simulink model "AvonGasTurbineDgTwin_fixed"  (R2024b)
settings: Solver=VariableStepAuto  StartTime=0  StopTime=7200  FixedStep=1  RelTol=1e-3  EnableMultiTasking=on
InitFcn:
  | warning off
model workspace (MAT data in the model file):
  FAULT_01_AirIntakeFilterFouling_enable = 1
  FAULT_02_CompBladeFouling_enable = 1
  FAULT_03_CompBladeDamage_enable = 1
  FAULT_04_CompSurgeStall_enable = 1
  FAULT_05_DiffuserDamage_enable = 1
  FAULT_06_IGVStuck_enable = 1
  FAULT_07_FuelPrssRegulatorStuck_enable = 1
  FAULT_08_FuelValveLeakage_enable = 1
  FAULT_09_FuelContamination_enable = 1
  FAULT_10_FuelLineBlockage_enable = 1
  FAULT_11_FuelPumpDegradation_enable = 1
  FAULT_12_FuelSupplyPressDrop_enable = 1
  FAULT_13_FGSupplyPressOscillation_enable = 1
  FAULT_14_FGValvePartialOpening_enable = 1
  FAULT_15_FGValveActuatorDelay_enable = 1
  FAULT_15_FuelPressReg_enable = 0
  FAULT_16_CombLinerDamage_enable = 1
  FAULT_16_FuelValveLeak_enable = 0
  FAULT_17_FuelNozzleClogging_enable = 1
  FAULT_18_CombustionFlameOscillation_enable = 1
  FAULT_19_CombustionInstability_enable = 1
  FAULT_20_HotGasPathTempIncrease_enable = 1
  FAULT_21_GGTurbFouling_enable = 1
  FAULT_22_GGTurbBladeDamage_enable = 1
  FAULT_23_GGNozzleBlockage_enable = 1
  FAULT_24_GGSealDegradation_enable = 1
  FAULT_25_GGInletPressureLoss_enable = 1
  FAULT_26_PTFouling_enable = 1
  FAULT_27_PTBladeDamage_enable = 1
  FAULT_28_PTNozzleDamage_enable = 1
  FAULT_29_PTSealDegradation_enable = 1
  FAULT_30_PTBearingWear_enable = 1
  FAULT_31_PTPowerLoss_enable = 1
  FAULT_32_PTStackBlockage_enable = 1
  FAULT_33_SensorEnhancement_enable = 1
  FAULT_34_SensorDegradation_enable = 1
  FAULT_35_SensorEnhanceStep_enable = 1
  FAULT_36_SensorDegradeStep_enable = 1
  FAULT_37_SensorFreez_enable = 1
  FAULT_38_GGSpeedSensor_enable = 1
  FAULT_39_PTSpeedSensor_enable = 1
  FAULT_40_FGSensorOffset_enable = 1
  FAULT_41_FGSensorDrift_enable = 1
  FAULT_42_ControlLoopOscillation_enable = 1
  GOV_GG_BASELINE = 10
  GOV_GG_DROOP_PCT = 0.04
  GOV_PT_BASELINE = 10
  GOV_PT_DROOP_PCT = 0.04
  SW_Manual_Switch1_enable = 1
  SW_Manual_Switch2_enable = 1
  SW_Manual_Switch3_enable = 1
  SW_Manual_Switch4_enable = 1
  SW_Manual_Switch_enable = 1
undefined symbols (not defined in the file or in its folder): ENV_ambient_moisture_pct, ENV_comp_inlet_press_kPa, ENV_FG_pressure_kPa, ENV_FG_temp_C, SP_POWER_CMD
libraries: slpidlib x3, simulink x2
(part 2 of 4)

== system AvonGasTurbineDgTwin_fixed/FAULT_06_IGVStuck ==
  IGV Pos : Inport
  FAULT_06_multiplier : FromWorkspace  VariableName=FAULT_06_multiplier  SampleTime=-1
  Mux : Mux  Inputs=2
  Product : Product
  Scope{,1..3} (4 alike) : Scope  Commented=on
  Out1 : Outport
  wires:
  FAULT_06_multiplier/1 -> Product/1, Scope/1
  IGV Pos/1 -> Scope1/1, Mux/2, Product/2
  Product/1 -> Mux/1, Scope2/1, Out1/1
  Mux/1 -> Scope3/1

== system AvonGasTurbineDgTwin_fixed/FAULT_15_FuelPressReg ==
  In1 : Inport
  FAULT_15_multiplier : FromWorkspace  VariableName=FAULT_15_multiplier  SampleTime=-1
  Mux : Mux  Inputs=2
  Product : Product
  Scope{,1..3} (4 alike) : Scope  Commented=on
  Out1 : Outport
  wires:
  FAULT_15_multiplier/1 -> Product/1, Scope/1
  In1/1 -> Scope1/1, Mux/2, Product/2
  Product/1 -> Mux/1, Scope2/1, Out1/1
  Mux/1 -> Scope3/1

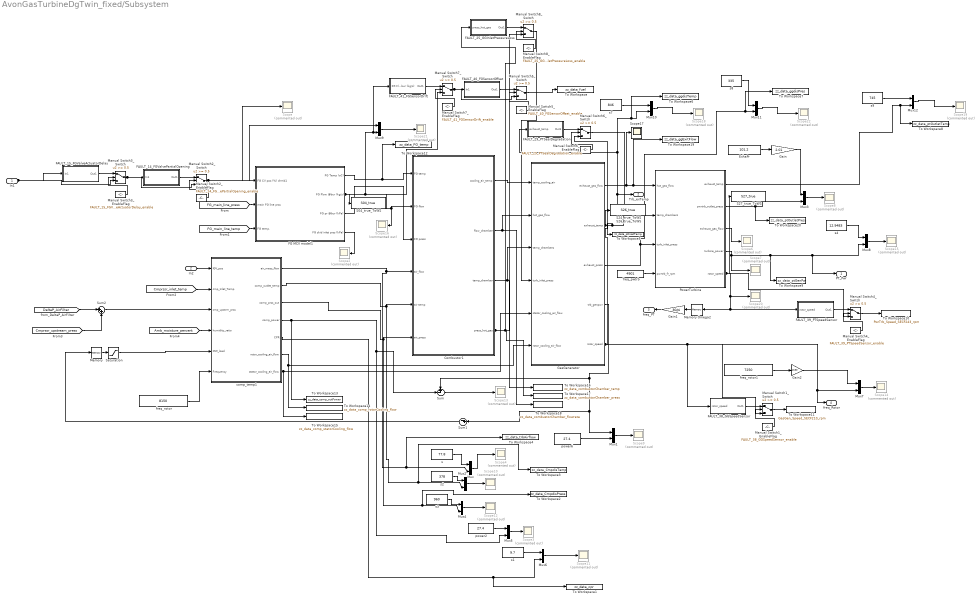
== system AvonGasTurbineDgTwin_fixed/Subsystem ==
  In1 : Inport
  In2 : Inport  Port=2
  Combustor1 : Subsystem
  ExhaPr : Constant  Value=101.2
  FAULT_14_FGValvePartialOpening : Subsystem
  FAULT_15_FGValveActuatorDelay : Subsystem
  FAULT_25_GGInletPressureLoss : Subsystem
  FAULT_29_PTSealDegradation : Subsystem
  FAULT_38_GGSpeedSensor : Subsystem
  FAULT_39_PTSpeedSensor : Subsystem
  FAULT_40_FGSensorOffset : Subsystem
  FAULT_41_FGSensorDrift : Subsystem
  FG MCV model1 : Subsystem
  Gain : Gain  Gain=2.01
  Gain1 : Gain  Gain=30/pi
  Gain2 : Gain  Gain=pi/30
  GasGenerator : Subsystem
  Manual Switch1_EnableFlag : Constant  Value=FAULT_38_GGSpeedSensor_enable
  Manual Switch1_Switch : Switch  Threshold=0.5  SaturateOnIntegerOverflow=off  InputSameDT=off
  Manual Switch2_EnableFlag : Constant  Value=FAULT_14_FGValvePartialOpening_enable
  Manual Switch2_Switch : Switch  Threshold=0.5  SaturateOnIntegerOverflow=off  InputSameDT=off
  Manual Switch3_EnableFlag : Constant  Value=FAULT_15_FGValveActuatorDelay_enable
  Manual Switch3_Switch : Switch  Threshold=0.5  SaturateOnIntegerOverflow=off  InputSameDT=off
  Manual Switch4_EnableFlag : Constant  Value=FAULT_39_PTSpeedSensor_enable
  Manual Switch4_Switch : Switch  Threshold=0.5  SaturateOnIntegerOverflow=off  InputSameDT=off
  Manual Switch5_EnableFlag : Constant  Value=FAULT_40_FGSensorOffset_enable
  Manual Switch5_Switch : Switch  Threshold=0.5  SaturateOnIntegerOverflow=off  InputSameDT=off
  Manual Switch6_EnableFlag : Constant  Value=FAULT_29_PTSealDegradation_enable
  Manual Switch6_Switch : Switch  Threshold=0.5  SaturateOnIntegerOverflow=off  InputSameDT=off
  Manual Switch7_EnableFlag : Constant  Value=FAULT_41_FGSensorDrift_enable
  Manual Switch7_Switch : Switch  Threshold=0.5  SaturateOnIntegerOverflow=off  InputSameDT=off
  Manual Switch8_EnableFlag : Constant  Value=FAULT_25_GGInletPressureLoss_enable
  Manual Switch8_Switch : Switch  Threshold=0.5  SaturateOnIntegerOverflow=off  InputSameDT=off
  Memory : Memory  InitialCondition=28.945
  Memory Omega2 : Memory  InitialCondition=pi/30*4901
  Mux{,1..12} (13 alike) : Mux  Inputs=2
  PowerTurbine : Subsystem
  S04_true_ToWS : ToWorkspace  VariableName=S04_true  SampleTime=-1
  S24_true_ToWS : ToWorkspace  VariableName=S24_true  SampleTime=-1
  S26_true_ToWS : ToWorkspace  VariableName=S26_true  SampleTime=-1
  S27_true_ToWS : ToWorkspace  VariableName=S27_true  SampleTime=-1
  Saturation : Saturate  UpperLimit=40  LowerLimit=1
  Scope{,2..4,6..16,18..22} (20 alike) : Scope  Commented=on
  Scope17 : Scope
  Sum : Sum  Inputs=+-|
  Sum1 : Sum  Inputs=-+|
  Sum2 : Sum  Inputs=|++
  To Workspace : ToWorkspace  VariableName=zz_data_fuel  SampleTime=0.2
  To Workspace1 : ToWorkspace  VariableName=zz_data_cpr  SampleTime=0.2
  To Workspace10 : ToWorkspace  VariableName=PwrTrb_Speed_SECF243_rpm  SampleTime=0.2
  To Workspace11 : ToWorkspace  VariableName=GasGen_Speed_SECF210_rpm  SampleTime=0.2
  To Workspace12 : ToWorkspace  VariableName=zz_data_FG_temp  SampleTime=0.2
  To Workspace13 : ToWorkspace  VariableName=zz_data_comp_outPower  SampleTime=0.2
  To Workspace14 : ToWorkspace  VariableName=zz_data_comp_rotorCooling_flow  SampleTime=0.2
  To Workspace15 : ToWorkspace  VariableName=zz_data_comp_statorCooling_flow  SampleTime=0.2
  To Workspace16 : ToWorkspace  VariableName=zz_data_combustorChamber_temp  SampleTime=0.2
  To Workspace17 : ToWorkspace  VariableName=zz_data_combustorChamber_press  SampleTime=0.2
  To Workspace18 : ToWorkspace  VariableName=zz_data_combustorChamber_flowrate  SampleTime=0.2
  To Workspace19 : ToWorkspace  VariableName=zz_data_ggExitFlow  SampleTime=0.2
  To Workspace2 : ToWorkspace  VariableName=zz_data_CmpdisPress  SampleTime=0.2
  To Workspace20 : ToWorkspace  VariableName=zz_data_ptOutletPress  SampleTime=0.2
  To Workspace3 : ToWorkspace  VariableName=zz_data_CmpdisTemp  SampleTime=0.2
  To Workspace4 : ToWorkspace  VariableName=zz_data_trbAirflow  SampleTime=0.2
  To Workspace5 : ToWorkspace  VariableName=zz_data_ptInletTemp  SampleTime=0.2
  To Workspace6 : ToWorkspace  VariableName=zz_data_ggdisTemp  SampleTime=0.2
  To Workspace7 : ToWorkspace  VariableName=zz_data_ggdisPres  SampleTime=0.2
  To Workspace8 : ToWorkspace  VariableName=zz_data_ptOutletTemp  SampleTime=0.2
  To Workspace9 : ToWorkspace  VariableName=zz_data_ptGenPw  SampleTime=0.2
  comp_temp1 : Subsystem
  freq_pwtrb : Constant  Value=4901
  freq_rotor : Constant  Value=8150
  freq_rotor1 : Constant  Value=7250
  power2 : Constant  Value=27.4
  power6 : Constant  Value=27.4
  s : Constant  Value=77.8
  s1 : Constant  Value=9.7
  s2 : Constant  Value=378
  s3 : Constant  Value=960
  s4 : Constant  Value=12.9483
  s7 : Constant  Value=846
  s8 : Constant  Value=335
  s9 : Constant  Value=745
  PT_Pwr : Outport
  Trb_exTemp : Outport  Port=2
  freq_PT : Outport  Port=3
  freq_Rotor : Outport  Port=4
  wires:
  Gain1/1 -> freq_PT/1
  GasGenerator/2(exhaust_temp) -> To Workspace5/1, Trb_exTemp/1, To Workspace6/1, Mux10/2, FAULT_29_PTSealDegradation/1(exhaust_temp), Manual Switch6_Switch/3, S26_true_ToWS/1
  [Amb_moisture_percent] -> comp_temp1/4(humidity_ratio)
  freq_rotor/1 -> comp_temp1/6(Frequency)
  In2/1 -> comp_temp1/1(IGV_pos)
  PowerTurbine/3(exhaust_gas_flow) -> Scope6/1
  Memory/1 -> Saturation/1
  comp_temp1/3(comp_prss_out) -> To Workspace2/1, Mux4/2, Combustor1/6(air_press)
  FG MCV model1/2(FG Flow @bur (kg/s)) -> Mux9/2, FAULT_41_FGSensorDrift/1(FG Flow @bur (kg/s)), Scope16/1, Combustor1/2(FG flow), Manual Switch7_Switch/3, S04_true_ToWS/1
  Combustor1/2(flow_chamber) -> To Workspace18/1, GasGenerator/2(hot_gas_flow)
  comp_temp1/4(comp_power) -> To Workspace13/1, Mux5/2, Sum/2
  Mux1/1 -> Scope9/1
  Mux6/1 -> Scope11/1
  comp_temp1/5(CPR) -> To Workspace1/1, Mux6/2
  Mux4/1 -> Scope12/1
  FG MCV model1/1(FG Temp (oC)) -> To Workspace12/1, Combustor1/1(FG temp)
  Mux2/1 -> Scope10/1
  [FG_main_line_press] -> FG MCV model1/2(main FG line prss)
  ExhaPr/1 -> Gain/1
  Combustor1/1(cooling_air_temp) -> GasGenerator/1(temp_cooling_air)
  FG MCV model1/3(FG pr @bur (kPa)) -> Combustor1/3(FG press)
  GasGenerator/3(exhaust_press) -> To Workspace7/1, Mux11/2, PowerTurbine/3(turb_inlet_press)
  Combustor1/3(temp_chamber) -> To Workspace16/1, GasGenerator/3(temp_chambers)
  FG MCV model1/4(FG skid inlet prss (kPa)) -> Scope2/1
  GasGenerator/1(exhaust_gas_flow) -> Scope17/1, To Workspace19/1, PowerTurbine/1(hot_gas_flow)
  PowerTurbine/2(pwrtrb_outlet_press) -> To Workspace20/1, Mux3/2
  power6/1 -> Mux1/2
  Gain/1 -> Mux3/1
  Mux3/1 -> Scope8/1
  comp_temp1/1(air_mass_flow) -> To Workspace4/1, Mux/2, Combustor1/4(air_flow)
  PowerTurbine/1(exhaust_temp) -> To Workspace8/1, Mux12/2
  comp_temp1/2(comp_outlet_temp) -> To Workspace3/1, Mux2/2, Combustor1/5(air temp)
  Mux8/1 -> Scope15/1
  Mux7/1 -> Scope14/1
  In1/1 -> FAULT_15_FGValveActuatorDelay/1(In1), Manual Switch3_Switch/3
  PowerTurbine/4(turbine_power) -> To Workspace9/1, PT_Pwr/1, Mux8/2, Scope7/1
  comp_temp1/7(stator_cooling_air_flow) -> GasGenerator/5(stator_cooling_air_flow), To Workspace15/1
  [Cmprssr_inlet_temp] -> comp_temp1/2(cmp_Inlet_Temp)
  Mux11/1 -> Scope22/1
  s2/1 -> Mux2/1
  Sum1/1 -> Memory/1
  Mux9/1 -> Scope21/1
  Mux/1 -> Scope4/1
  s/1 -> Mux/1
  s7/1 -> Mux10/1
  s1/1 -> Mux6/1
  Mux10/1 -> Scope18/1
  Mux5/1 -> Scope3/1
  Sum/1 -> Scope13/1
  GasGenerator/5(rotor_speed) -> freq_Rotor/1, Mux7/2, FAULT_38_GGSpeedSensor/1(rotor_speed), Manual Switch1_Switch/3, S24_true_ToWS/1
  comp_temp1/6(rotor_cooling_air_flow) -> GasGenerator/6(rotor_cooling_air_flow), To Workspace14/1
  s3/1 -> Mux4/1
  freq_pwtrb/1 -> PowerTurbine/4(pwrtrb_fr_rpm)
  power2/1 -> Mux5/1
  PowerTurbine/5(rotor_speed) -> Memory Omega2/1, FAULT_39_PTSpeedSensor/1(rotor_speed), Scope20/1, Manual Switch4_Switch/3, S27_true_ToWS/1
  Gain2/1 -> Mux7/1
  Saturation/1 -> comp_temp1/5(MW_load)
  Memory Omega2/1 -> Gain1/1
  freq_rotor1/1 -> Gain2/1
  GasGenerator/4(trb_genpwr) -> Sum/1, Sum1/2, Mux1/1
  s4/1 -> Mux8/1
  s9/1 -> Mux12/1
  s8/1 -> Mux11/1
  Mux12/1 -> Scope19/1
  [FG_main_line_temp] -> FG MCV model1/3(FG temp.)
  [DeltaP_AirFilter] -> Sum2/1
  [Cmprssr_upstream_press] -> Sum2/2
  Sum2/1 -> comp_temp1/3(cmp_upstrm_prss)
  Combustor1/4(press_hot_gas) -> To Workspace17/1, FAULT_25_GGInletPressureLoss/1(press_hot_gas), Manual Switch8_Switch/3
  FAULT_38_GGSpeedSensor/1(Out1) -> Manual Switch1_Switch/1
  Manual Switch1_EnableFlag/1 -> Manual Switch1_Switch/2
  Manual Switch1_Switch/1 -> To Workspace11/1
  FAULT_14_FGValvePartialOpening/1(Out1) -> Manual Switch2_Switch/1
  Manual Switch2_EnableFlag/1 -> Manual Switch2_Switch/2
  Manual Switch2_Switch/1 -> FG MCV model1/1(FG CV pos (%) chmb1), Scope/1, Mux9/1
  FAULT_15_FGValveActuatorDelay/1(Out1) -> Manual Switch3_Switch/1
  Manual Switch3_EnableFlag/1 -> Manual Switch3_Switch/2
  Manual Switch3_Switch/1 -> Manual Switch2_Switch/3, FAULT_14_FGValvePartialOpening/1(In1)
  FAULT_39_PTSpeedSensor/1(Out1) -> Manual Switch4_Switch/1
  Manual Switch4_EnableFlag/1 -> Manual Switch4_Switch/2
  Manual Switch4_Switch/1 -> To Workspace10/1
  FAULT_40_FGSensorOffset/1(Out1) -> Manual Switch5_Switch/1
  Manual Switch5_EnableFlag/1 -> Manual Switch5_Switch/2
  Manual Switch5_Switch/1 -> To Workspace/1
  FAULT_29_PTSealDegradation/1(Out1) -> Manual Switch6_Switch/1
  Manual Switch6_EnableFlag/1 -> Manual Switch6_Switch/2
  Manual Switch6_Switch/1 -> PowerTurbine/2(temp_chambers)
  FAULT_41_FGSensorDrift/1(Out1) -> Manual Switch7_Switch/1
  Manual Switch7_EnableFlag/1 -> Manual Switch7_Switch/2
  Manual Switch7_Switch/1 -> Manual Switch5_Switch/3, FAULT_40_FGSensorOffset/1(In1)
  FAULT_25_GGInletPressureLoss/1(Out1) -> Manual Switch8_Switch/1
  Manual Switch8_EnableFlag/1 -> Manual Switch8_Switch/2
  Manual Switch8_Switch/1 -> GasGenerator/4(turb_inlet_press)

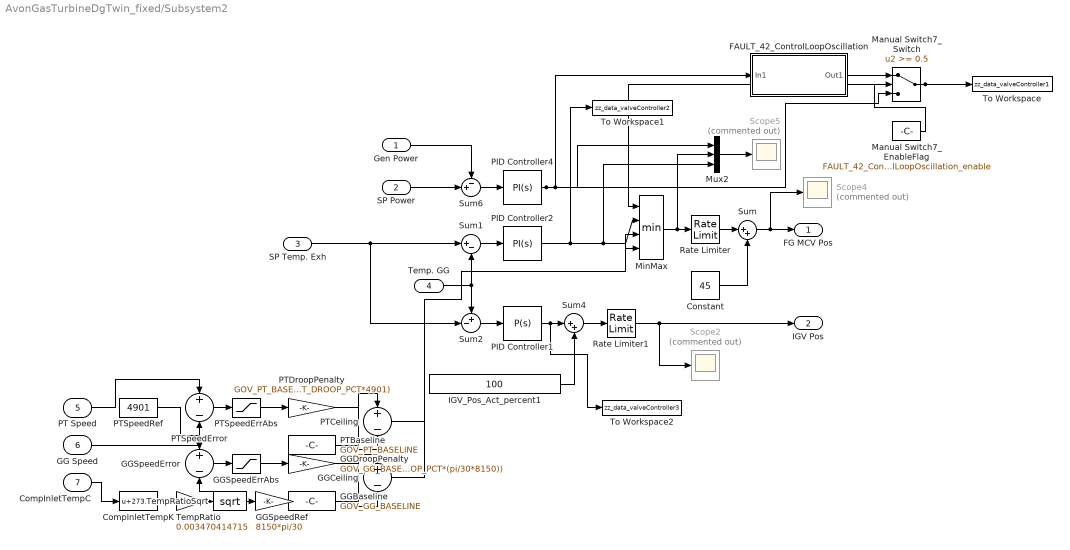
== system AvonGasTurbineDgTwin_fixed/Subsystem2 ==
  Gen Power : Inport
  SP Power : Inport  Port=2
  SP Temp. Exh : Inport  Port=3
  Temp. GG : Inport  Port=4
  PT Speed : Inport  Port=5
  GG Speed : Inport  Port=6
  CompInletTempC : Inport  Port=7
  CompInletTempK : Bias  Bias=273.15  SaturateOnIntegerOverflow=off
  Constant : Constant  Value=45
  FAULT_42_ControlLoopOscillation : Subsystem
  GGBaseline : Constant  Value=GOV_GG_BASELINE
  GGCeiling : Sum  Inputs=+-
  GGDroopPenalty : Gain  Gain=GOV_GG_BASELINE/(GOV_GG_DROOP_PCT*(pi/30*8150))
  GGSpeedErrAbs : Saturate  UpperLimit=Inf  LowerLimit=0
  GGSpeedError : Sum  Inputs=+-
  GGSpeedRef : Gain  Gain=8150*pi/30
  IGV_Pos_Act_percent1 : Constant  Value=100
  Manual Switch7_EnableFlag : Constant  Value=FAULT_42_ControlLoopOscillation_enable
  Manual Switch7_Switch : Switch  Threshold=0.5  SaturateOnIntegerOverflow=off  InputSameDT=off
  MinMax : MinMax  Inputs=4
  Mux2 : Mux  Inputs=3
  PID Controller1 : slpidlib/PID Controller  Controller=P  Form=Ideal  TimeDomain=Continuous-time  UseExternalTs=off  SampleTime=-1  IntegratorMethod=Forward Euler  FilterMethod=Forward Euler  ControllerParametersSource=internal  P=0.1  I=0.180070827922895  UseKiTs=off  D=0  UseExternalDerivativeSource=off  N=100  UseFilter=on  TunerSelectOption=Transfer Function Based (PID Tuner App)  InitialConditionSource=internal  InitialConditionForIntegrator=0  InitialConditionForFilter=0  DifferentiatorICPrevScaledInput=0  ExternalReset=none  TrackingMode=off  Kt=1  LimitOutput=on  SatLimitsSource=internal  UpperSaturationLimit=15  LowerSaturationLimit=-100  LinearizeAsGain=on  AntiWindupMode=back-calculation  Kb=0.2  LimitIntegrator=off  UpperIntegratorSaturationLimit=inf  LowerIntegratorSaturationLimit=-inf  POutMin=[]  POutMax=[]  IOutMin=[]  IOutMax=[]  DOutMin=[]  DOutMax=[]  NOutMin=[]  NOutMax=[]  SumOutMin=[]  SumOutMax=[]  SaturationOutMin=[]  SaturationOutMax=[]  PParamMin=[]  PParamMax=[]  IParamMin=[]  IParamMax=[]  DParamMin=[]  DParamMax=[]  NParamMin=[]  NParamMax=[]  KbParamMin=[]  KbParamMax=[]  KtParamMin=[]  KtParamMax=[]  KbOutMin=[]  KbOutMax=[]  KtOutMin=[]  KtOutMax=[]  IntegratorOutMin=[]  IntegratorOutMax=[]  FilterOutMin=[]  FilterOutMax=[]  SumI1OutMin=[]  SumI1OutMax=[]  SumI2OutMin=[]  SumI2OutMax=[]  SumI3OutMin=[]  SumI3OutMax=[]  SumI4OutMin=[]  SumI4OutMax=[]  SumDOutMin=[]  SumDOutMax=[]  DifferentiatorOutMin=[]  DifferentiatorOutMax=[]  FilterDiffOutCoefMin=[]  FilterDiffOutCoefMax=[]  ReciprocalOutMin=[]  ReciprocalOutMax=[]  SumDenOutMin=[]  SumDenOutMax=[]  SumNumOutMin=[]  SumNumOutMax=[]  DivideOutMin=[]  DivideOutMax=[]  UdiffTsProdOutMin=[]  UdiffTsProdOutMax=[]  NTsProdOutMin=[]  NTsProdOutMax=[]  UintegralTsProdOutMin=[]  UintegralTsProdOutMax=[]  UngainTsProdOutMin=[]  UngainTsProdOutMax=[]  ClampingZeroOutDataTypeStr=Inherit: Inherit via back propagation  ClampingZeroOutMin=[]  ClampingZeroOutMax=[]  FilterDenConstantOutDataTypeStr=Inherit: Inherit via back propagation  FilterDenConstantOutMin=[]  FilterDenConstantOutMax=[]  PCopyOutDataTypeStr=Inherit: Inherit via back propagation  PCopyOutMin=[]  PCopyOutMax=[]  NCopyOutDataTypeStr=Inherit: Inherit via back propagation  NCopyOutMin=[]  NCopyOutMax=[]  IntegratorContinuousStateAttributes=''  IntegratorStateMustResolveToSignalObject=off  IntegratorRTWStateStorageClass=Auto  FilterContinuousStateAttributes=''  FilterStateMustResolveToSignalObject=off  FilterRTWStateStorageClass=Auto  ParallelPVariant=InternalParameters  IdealPVariant=Disabled  IVariant=Disabled  DVariant=Disabled  IntegratorVariant=Disabled  SatVariant=Enabled  AWVariant=Disabled  PCopyVariant=Disabled  TRVariant=Disabled  FdbkBlocksVariant=Forward  IdealPFdbkVariant=Disabled  SatFdbkVariant=Disabled  DerivativeFilterVariant=Disabled  NVariant=Disabled  NCopyVariant=Disabled_SignalSpec  FilterICVariant=Disabled  IntegratorICVariant=Disabled  ExternalResetVariant=Disabled  TRSumVariant=Passthrough  SumFdbkVariant=Disabled  SumVariant=Passthrough_P  TsampFilterVariant=InternalTs  TsampNgainVariant=Passthrough  TsampIntegralVariant=Disabled_SignalSpec  ExternalSaturationOutDataTypeStr=Inherit: Same as second input  DerivativeSourceVariant=Disabled  PreIntVariant=InternalPreInt
  PID Controller2 : slpidlib/PID Controller  Controller=PI  Form=Ideal  TimeDomain=Continuous-time  UseExternalTs=off  SampleTime=-1  IntegratorMethod=Forward Euler  FilterMethod=Forward Euler  ControllerParametersSource=internal  P=0.02  I=0.1  UseKiTs=off  D=0  UseExternalDerivativeSource=off  N=100  UseFilter=on  TunerSelectOption=Transfer Function Based (PID Tuner App)  InitialConditionSource=internal  InitialConditionForIntegrator=20  InitialConditionForFilter=0  DifferentiatorICPrevScaledInput=0  ExternalReset=none  TrackingMode=off  Kt=1  LimitOutput=on  SatLimitsSource=internal  UpperSaturationLimit=45  LowerSaturationLimit=-45  LinearizeAsGain=on  AntiWindupMode=back-calculation  Kb=0.2  LimitIntegrator=off  UpperIntegratorSaturationLimit=inf  LowerIntegratorSaturationLimit=-inf  POutMin=[]  POutMax=[]  IOutMin=[]  IOutMax=[]  DOutMin=[]  DOutMax=[]  NOutMin=[]  NOutMax=[]  SumOutMin=[]  SumOutMax=[]  SaturationOutMin=[]  SaturationOutMax=[]  PParamMin=[]  PParamMax=[]  IParamMin=[]  IParamMax=[]  DParamMin=[]  DParamMax=[]  NParamMin=[]  NParamMax=[]  KbParamMin=[]  KbParamMax=[]  KtParamMin=[]  KtParamMax=[]  KbOutMin=[]  KbOutMax=[]  KtOutMin=[]  KtOutMax=[]  IntegratorOutMin=[]  IntegratorOutMax=[]  FilterOutMin=[]  FilterOutMax=[]  SumI1OutMin=[]  SumI1OutMax=[]  SumI2OutMin=[]  SumI2OutMax=[]  SumI3OutMin=[]  SumI3OutMax=[]  SumI4OutMin=[]  SumI4OutMax=[]  SumDOutMin=[]  SumDOutMax=[]  DifferentiatorOutMin=[]  DifferentiatorOutMax=[]  FilterDiffOutCoefMin=[]  FilterDiffOutCoefMax=[]  ReciprocalOutMin=[]  ReciprocalOutMax=[]  SumDenOutMin=[]  SumDenOutMax=[]  SumNumOutMin=[]  SumNumOutMax=[]  DivideOutMin=[]  DivideOutMax=[]  UdiffTsProdOutMin=[]  UdiffTsProdOutMax=[]  NTsProdOutMin=[]  NTsProdOutMax=[]  UintegralTsProdOutMin=[]  UintegralTsProdOutMax=[]  UngainTsProdOutMin=[]  UngainTsProdOutMax=[]  ClampingZeroOutDataTypeStr=Inherit: Inherit via back propagation  ClampingZeroOutMin=[]  ClampingZeroOutMax=[]  FilterDenConstantOutDataTypeStr=Inherit: Inherit via back propagation  FilterDenConstantOutMin=[]  FilterDenConstantOutMax=[]  PCopyOutDataTypeStr=Inherit: Inherit via back propagation  PCopyOutMin=[]  PCopyOutMax=[]  NCopyOutDataTypeStr=Inherit: Inherit via back propagation  NCopyOutMin=[]  NCopyOutMax=[]  IntegratorContinuousStateAttributes=''  IntegratorStateMustResolveToSignalObject=off  IntegratorRTWStateStorageClass=Auto  FilterContinuousStateAttributes=''  FilterStateMustResolveToSignalObject=off  FilterRTWStateStorageClass=Auto  ParallelPVariant=Passthrough  IdealPVariant=InternalParameters  IVariant=InternalParameters  DVariant=Disabled  IntegratorVariant=Continuous  SatVariant=Enabled  AWVariant=BackCalculation  PCopyVariant=Disabled  TRVariant=Disabled  FdbkBlocksVariant=Forward  IdealPFdbkVariant=Disabled  SatFdbkVariant=Disabled  DerivativeFilterVariant=Disabled  NVariant=Disabled  NCopyVariant=Disabled_SignalSpec  FilterICVariant=Disabled  IntegratorICVariant=InternalICs  ExternalResetVariant=Disabled  TRSumVariant=Passthrough  SumFdbkVariant=Disabled  SumVariant=Sum_PI  TsampFilterVariant=InternalTs  TsampNgainVariant=Passthrough  TsampIntegralVariant=Disabled_SignalSpec  ExternalSaturationOutDataTypeStr=Inherit: Same as second input  DerivativeSourceVariant=Disabled  PreIntVariant=InternalPreInt
  PID Controller4 : slpidlib/PID Controller  Controller=PI  Form=Ideal  TimeDomain=Continuous-time  UseExternalTs=off  SampleTime=-1  IntegratorMethod=Forward Euler  FilterMethod=Forward Euler  ControllerParametersSource=internal  P=0.17  I=0.2  UseKiTs=off  D=0  UseExternalDerivativeSource=off  N=100  UseFilter=on  TunerSelectOption=Transfer Function Based (PID Tuner App)  InitialConditionSource=internal  InitialConditionForIntegrator=0  InitialConditionForFilter=0  DifferentiatorICPrevScaledInput=0  ExternalReset=none  TrackingMode=off  Kt=1  LimitOutput=on  SatLimitsSource=internal  UpperSaturationLimit=60  LowerSaturationLimit=-30  LinearizeAsGain=on  AntiWindupMode=back-calculation  Kb=0.2  LimitIntegrator=off  UpperIntegratorSaturationLimit=inf  LowerIntegratorSaturationLimit=-inf  POutMin=[]  POutMax=[]  IOutMin=[]  IOutMax=[]  DOutMin=[]  DOutMax=[]  NOutMin=[]  NOutMax=[]  SumOutMin=[]  SumOutMax=[]  SaturationOutMin=[]  SaturationOutMax=[]  PParamMin=[]  PParamMax=[]  IParamMin=[]  IParamMax=[]  DParamMin=[]  DParamMax=[]  NParamMin=[]  NParamMax=[]  KbParamMin=[]  KbParamMax=[]  KtParamMin=[]  KtParamMax=[]  KbOutMin=[]  KbOutMax=[]  KtOutMin=[]  KtOutMax=[]  IntegratorOutMin=[]  IntegratorOutMax=[]  FilterOutMin=[]  FilterOutMax=[]  SumI1OutMin=[]  SumI1OutMax=[]  SumI2OutMin=[]  SumI2OutMax=[]  SumI3OutMin=[]  SumI3OutMax=[]  SumI4OutMin=[]  SumI4OutMax=[]  SumDOutMin=[]  SumDOutMax=[]  DifferentiatorOutMin=[]  DifferentiatorOutMax=[]  FilterDiffOutCoefMin=[]  FilterDiffOutCoefMax=[]  ReciprocalOutMin=[]  ReciprocalOutMax=[]  SumDenOutMin=[]  SumDenOutMax=[]  SumNumOutMin=[]  SumNumOutMax=[]  DivideOutMin=[]  DivideOutMax=[]  UdiffTsProdOutMin=[]  UdiffTsProdOutMax=[]  NTsProdOutMin=[]  NTsProdOutMax=[]  UintegralTsProdOutMin=[]  UintegralTsProdOutMax=[]  UngainTsProdOutMin=[]  UngainTsProdOutMax=[]  ClampingZeroOutDataTypeStr=Inherit: Inherit via back propagation  ClampingZeroOutMin=[]  ClampingZeroOutMax=[]  FilterDenConstantOutDataTypeStr=Inherit: Inherit via back propagation  FilterDenConstantOutMin=[]  FilterDenConstantOutMax=[]  PCopyOutDataTypeStr=Inherit: Inherit via back propagation  PCopyOutMin=[]  PCopyOutMax=[]  NCopyOutDataTypeStr=Inherit: Inherit via back propagation  NCopyOutMin=[]  NCopyOutMax=[]  IntegratorContinuousStateAttributes=''  IntegratorStateMustResolveToSignalObject=off  IntegratorRTWStateStorageClass=Auto  FilterContinuousStateAttributes=''  FilterStateMustResolveToSignalObject=off  FilterRTWStateStorageClass=Auto  ParallelPVariant=Passthrough  IdealPVariant=InternalParameters  IVariant=InternalParameters  DVariant=Disabled  IntegratorVariant=Continuous  SatVariant=Enabled  AWVariant=BackCalculation  PCopyVariant=Disabled  TRVariant=Disabled  FdbkBlocksVariant=Forward  IdealPFdbkVariant=Disabled  SatFdbkVariant=Disabled  DerivativeFilterVariant=Disabled  NVariant=Disabled  NCopyVariant=Disabled_SignalSpec  FilterICVariant=Disabled  IntegratorICVariant=InternalICs  ExternalResetVariant=Disabled  TRSumVariant=Passthrough  SumFdbkVariant=Disabled  SumVariant=Sum_PI  TsampFilterVariant=InternalTs  TsampNgainVariant=Passthrough  TsampIntegralVariant=Disabled_SignalSpec  ExternalSaturationOutDataTypeStr=Inherit: Same as second input  DerivativeSourceVariant=Disabled  PreIntVariant=InternalPreInt
  PTBaseline : Constant  Value=GOV_PT_BASELINE
  PTCeiling : Sum  Inputs=+-
  PTDroopPenalty : Gain  Gain=GOV_PT_BASELINE/(GOV_PT_DROOP_PCT*4901)
  PTSpeedErrAbs : Saturate  UpperLimit=Inf  LowerLimit=0
  PTSpeedError : Sum  Inputs=+-
  PTSpeedRef : Constant  Value=4901
  Rate Limiter : RateLimiter  RisingSlewLimit=0.1  FallingSlewLimit=-0.1  SampleTimeMode=inherited  InitialCondition=45
  Rate Limiter1 : RateLimiter  RisingSlewLimit=0.1  FallingSlewLimit=-0.1  SampleTimeMode=inherited  InitialCondition=45
  Scope2 : Scope  Commented=on
  Scope4 : Scope  Commented=on
  Scope5 : Scope  Commented=on
  Sum : Sum  Inputs=|++
  Sum1 : Sum  Inputs=|+-
  Sum2 : Sum  Inputs=+-|
  Sum4 : Sum  Inputs=|++
  Sum6 : Sum  Inputs=-+|
  TempRatio : Gain  Gain=0.003470414715
  TempRatioSqrt : Math  Operator=sqrt
  To Workspace : ToWorkspace  VariableName=zz_data_valveController1  SampleTime=0.2
  To Workspace1 : ToWorkspace  VariableName=zz_data_valveController2  SampleTime=0.2
  To Workspace2 : ToWorkspace  VariableName=zz_data_valveController3  SampleTime=0.2
  FG MCV Pos : Outport
  IGV Pos : Outport  Port=2
  wires:
  Gen Power/1 -> Sum6/1
  MinMax/1 -> Mux2/2, Rate Limiter/1
  Mux2/1 -> Scope5/1
  Sum6/1 -> PID Controller4/1
  PID Controller4/1 -> FAULT_42_ControlLoopOscillation/1(In1), Mux2/1, Manual Switch7_Switch/3
  SP Temp. Exh/1 -> Sum2/2, Sum1/1
  Temp. GG/1 -> Sum2/1, Sum1/2
  Sum/1 -> FG MCV Pos/1, Scope4/1
  Constant/1 -> Sum/2
  Sum2/1 -> PID Controller1/1
  IGV_Pos_Act_percent1/1 -> Sum4/2
  PID Controller1/1 -> To Workspace2/1, Sum4/1
  Sum4/1 -> Rate Limiter1/1
  PID Controller2/1 -> MinMax/2, Mux2/3, To Workspace1/1
  Rate Limiter1/1 -> IGV Pos/1, Scope2/1
  Rate Limiter/1 -> Sum/1
  SP Power/1 -> Sum6/2
  Sum1/1 -> PID Controller2/1
  PT Speed/1 -> PTSpeedError/1
  PTSpeedRef/1 -> PTSpeedError/2
  PTSpeedError/1 -> PTSpeedErrAbs/1
  PTSpeedErrAbs/1 -> PTDroopPenalty/1
  PTBaseline/1 -> PTCeiling/1
  PTDroopPenalty/1 -> PTCeiling/2
  CompInletTempC/1 -> CompInletTempK/1
  CompInletTempK/1 -> TempRatio/1
  TempRatio/1 -> TempRatioSqrt/1
  TempRatioSqrt/1 -> GGSpeedRef/1
  GG Speed/1 -> GGSpeedError/1
  GGSpeedRef/1 -> GGSpeedError/2
  GGSpeedError/1 -> GGSpeedErrAbs/1
  GGSpeedErrAbs/1 -> GGDroopPenalty/1
  GGBaseline/1 -> GGCeiling/1
  GGDroopPenalty/1 -> GGCeiling/2
  PTCeiling/1 -> MinMax/3
  GGCeiling/1 -> MinMax/4
  FAULT_42_ControlLoopOscillation/1(Out1) -> Manual Switch7_Switch/1
  Manual Switch7_EnableFlag/1 -> Manual Switch7_Switch/2
  Manual Switch7_Switch/1 -> To Workspace/1, MinMax/1

== system AvonGasTurbineDgTwin_fixed/Subsystem/Combustor1 ==
  FG temp : Inport
  FG flow : Inport  Port=2
  FG press : Inport  Port=3
  air_flow : Inport  Port=4
  air temp : Inport  Port=5
  air_press : Inport  Port=6
  FAULT_16_CombLinerDamage : Subsystem
  FAULT_17_FuelNozzleClogging : Subsystem
  FAULT_18_CombustionFlameOscillation : Subsystem
  FAULT_19_CombustionInstability : Subsystem
  FAULT_20_HotGasPathTempIncrease : Subsystem
  Manual Switch1_EnableFlag : Constant  Value=FAULT_17_FuelNozzleClogging_enable
  Manual Switch1_Switch : Switch  Threshold=0.5  SaturateOnIntegerOverflow=off  InputSameDT=off
  Manual Switch2_EnableFlag : Constant  Value=FAULT_20_HotGasPathTempIncrease_enable
  Manual Switch2_Switch : Switch  Threshold=0.5  SaturateOnIntegerOverflow=off  InputSameDT=off
  Manual Switch3_EnableFlag : Constant  Value=FAULT_18_CombustionFlameOscillation_enable
  Manual Switch3_Switch : Switch  Threshold=0.5  SaturateOnIntegerOverflow=off  InputSameDT=off
  Manual Switch4_EnableFlag : Constant  Value=FAULT_19_CombustionInstability_enable
  Manual Switch4_Switch : Switch  Threshold=0.5  SaturateOnIntegerOverflow=off  InputSameDT=off
  Manual Switch7_EnableFlag : Constant  Value=FAULT_16_CombLinerDamage_enable
  Manual Switch7_Switch : Switch  Threshold=0.5  SaturateOnIntegerOverflow=off  InputSameDT=off
  Scope{1..4} (4 alike) : Scope
  combustion chamber 1 : Subsystem
  cooling_air_temp : Outport
  flow_chamber : Outport  Port=2
  temp_chamber : Outport  Port=3
  press_hot_gas : Outport  Port=4
  wires:
  FG press/1 -> combustion chamber 1/2(FG press)
  FG temp/1 -> combustion chamber 1/3(FG temp)
  air_press/1 -> combustion chamber 1/6(air_press)
  air temp/1 -> Scope2/1, cooling_air_temp/1, combustion chamber 1/5(air_temp)
  combustion chamber 1/2(flow) -> Scope3/1, flow_chamber/1
  combustion chamber 1/3(Gas_press) -> press_hot_gas/1
  air_flow/1 -> FAULT_16_CombLinerDamage/1(air_flow), Manual Switch7_Switch/3
  FG flow/1 -> FAULT_17_FuelNozzleClogging/1(FG flow), Manual Switch1_Switch/3
  combustion chamber 1/1(temp chamber 1) -> FAULT_18_CombustionFlameOscillation/1(temp chamber 1), Manual Switch3_Switch/3
  FAULT_17_FuelNozzleClogging/1(Out1) -> Manual Switch1_Switch/1
  Manual Switch1_EnableFlag/1 -> Manual Switch1_Switch/2
  Manual Switch1_Switch/1 -> combustion chamber 1/1(Fg flow)
  FAULT_20_HotGasPathTempIncrease/1(Out1) -> Manual Switch2_Switch/1
  Manual Switch2_EnableFlag/1 -> Manual Switch2_Switch/2
  Manual Switch2_Switch/1 -> temp_chamber/1, Scope1/1
  FAULT_18_CombustionFlameOscillation/1(Out1) -> Manual Switch3_Switch/1
  Manual Switch3_EnableFlag/1 -> Manual Switch3_Switch/2
  Manual Switch3_Switch/1 -> FAULT_19_CombustionInstability/1(In1), Manual Switch4_Switch/3
  FAULT_19_CombustionInstability/1(Out1) -> Manual Switch4_Switch/1
  Manual Switch4_EnableFlag/1 -> Manual Switch4_Switch/2
  Manual Switch4_Switch/1 -> Manual Switch2_Switch/3, FAULT_20_HotGasPathTempIncrease/1(In1)
  FAULT_16_CombLinerDamage/1(Out1) -> Manual Switch7_Switch/1
  Manual Switch7_EnableFlag/1 -> Manual Switch7_Switch/2
  Manual Switch7_Switch/1 -> combustion chamber 1/4(air flow), Scope4/1

== system AvonGasTurbineDgTwin_fixed/Subsystem/FAULT_14_FGValvePartialOpening ==
  In1 : Inport
  FAULT_14_multiplier : FromWorkspace  VariableName=FAULT_14_multiplier  SampleTime=-1
  Mux : Mux  Inputs=2
  Product : Product
  Scope{,1..3} (4 alike) : Scope  Commented=on
  Out1 : Outport
  wires:
  FAULT_14_multiplier/1 -> Product/1, Scope/1
  In1/1 -> Scope1/1, Mux/2, Product/2
  Product/1 -> Mux/1, Scope2/1, Out1/1
  Mux/1 -> Scope3/1

== system AvonGasTurbineDgTwin_fixed/Subsystem/FAULT_15_FGValveActuatorDelay ==
  In1 : Inport
  FAULT_15_multiplier : FromWorkspace  VariableName=FAULT_15_multiplier  SampleTime=-1
  Mux : Mux  Inputs=2
  Product : Product
  Scope{,1..3} (4 alike) : Scope  Commented=on
  Out1 : Outport
  wires:
  FAULT_15_multiplier/1 -> Product/1, Scope/1
  In1/1 -> Scope1/1, Mux/2, Product/2
  Product/1 -> Mux/1, Scope2/1, Out1/1
  Mux/1 -> Scope3/1

== system AvonGasTurbineDgTwin_fixed/Subsystem/FAULT_25_GGInletPressureLoss ==
  press_hot_gas : Inport
  FAULT_25_multiplier : FromWorkspace  VariableName=FAULT_25_multiplier  SampleTime=-1
  Mux : Mux  Inputs=2
  Product : Product
  Scope{,1..3} (4 alike) : Scope  Commented=on
  Out1 : Outport
  wires:
  FAULT_25_multiplier/1 -> Product/1, Scope/1
  press_hot_gas/1 -> Scope1/1, Mux/2, Product/2
  Product/1 -> Mux/1, Scope2/1, Out1/1
  Mux/1 -> Scope3/1

== system AvonGasTurbineDgTwin_fixed/Subsystem/FAULT_29_PTSealDegradation ==
  exhaust_temp : Inport
  FAULT_29_multiplier : FromWorkspace  VariableName=FAULT_29_multiplier  SampleTime=-1
  Mux : Mux  Inputs=2
  Product : Product
  Scope{,1..3} (4 alike) : Scope  Commented=on
  Out1 : Outport
  wires:
  FAULT_29_multiplier/1 -> Product/1, Scope/1
  exhaust_temp/1 -> Scope1/1, Mux/2, Product/2
  Product/1 -> Mux/1, Scope2/1, Out1/1
  Mux/1 -> Scope3/1

== system AvonGasTurbineDgTwin_fixed/Subsystem/FAULT_38_GGSpeedSensor ==
  rotor_speed : Inport
  FAULT_38_multiplier : FromWorkspace  VariableName=FAULT_38_multiplier  SampleTime=-1
  Mux : Mux  Inputs=2
  Product : Product
  Scope{,1..3} (4 alike) : Scope  Commented=on
  Out1 : Outport
  wires:
  FAULT_38_multiplier/1 -> Product/1, Scope/1
  rotor_speed/1 -> Scope1/1, Mux/2, Product/2
  Product/1 -> Mux/1, Scope2/1, Out1/1
  Mux/1 -> Scope3/1

== system AvonGasTurbineDgTwin_fixed/Subsystem/FAULT_39_PTSpeedSensor ==
  rotor_speed : Inport
  FAULT_39_multiplier : FromWorkspace  VariableName=FAULT_39_multiplier  SampleTime=-1
  Mux : Mux  Inputs=2
  Product : Product
  Scope{,1..3} (4 alike) : Scope  Commented=on
  Out1 : Outport
  wires:
  FAULT_39_multiplier/1 -> Product/1, Scope/1
  rotor_speed/1 -> Scope1/1, Mux/2, Product/2
  Product/1 -> Mux/1, Scope2/1, Out1/1
  Mux/1 -> Scope3/1

== system AvonGasTurbineDgTwin_fixed/Subsystem/FAULT_40_FGSensorOffset ==
  In1 : Inport
  FAULT_40_multiplier : FromWorkspace  VariableName=FAULT_40_multiplier  SampleTime=-1
  Mux : Mux  Inputs=2
  Product : Product
  Scope{,1..3} (4 alike) : Scope  Commented=on
  Out1 : Outport
  wires:
  FAULT_40_multiplier/1 -> Product/1, Scope/1
  In1/1 -> Scope1/1, Mux/2, Product/2
  Product/1 -> Mux/1, Scope2/1, Out1/1
  Mux/1 -> Scope3/1

== system AvonGasTurbineDgTwin_fixed/Subsystem/FAULT_41_FGSensorDrift ==
  FG Flow @bur (kg/s) : Inport
  FAULT_41_multiplier : FromWorkspace  VariableName=FAULT_41_multiplier  SampleTime=-1
  Mux : Mux  Inputs=2
  Product : Product
  Scope{,1..3} (4 alike) : Scope  Commented=on
  Out1 : Outport
  wires:
  FAULT_41_multiplier/1 -> Product/1, Scope/1
  FG Flow @bur (kg/s)/1 -> Scope1/1, Mux/2, Product/2
  Product/1 -> Mux/1, Scope2/1, Out1/1
  Mux/1 -> Scope3/1

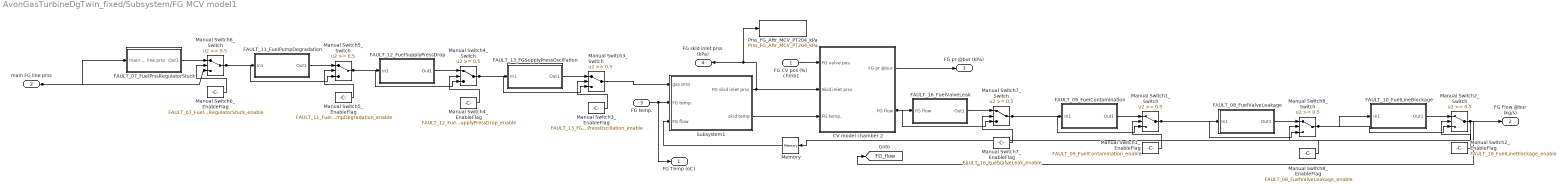
== system AvonGasTurbineDgTwin_fixed/Subsystem/FG MCV model1 ==
  FG CV pos (%) chmb1 : Inport
  main FG line prss : Inport  Port=2
  FG temp. : Inport  Port=3
  " Memory " : Memory  InitialCondition=1.9
  CV model chamber 2 : Subsystem
  FAULT_07_FuelPrssRegulatorStuck : Subsystem
  FAULT_08_FuelValveLeakage : Subsystem
  FAULT_09_FuelContamination : Subsystem
  FAULT_10_FuelLineBlockage : Subsystem
  FAULT_11_FuelPumpDegradation : Subsystem
  FAULT_12_FuelSupplyPressDrop : Subsystem
  FAULT_13_FGSupplyPressOscillation : Subsystem
  FAULT_16_FuelValveLeak : Subsystem
  Manual Switch1_EnableFlag : Constant  Value=FAULT_09_FuelContamination_enable
  Manual Switch1_Switch : Switch  Threshold=0.5  SaturateOnIntegerOverflow=off  InputSameDT=off
  Manual Switch2_EnableFlag : Constant  Value=FAULT_10_FuelLineBlockage_enable
  Manual Switch2_Switch : Switch  Threshold=0.5  SaturateOnIntegerOverflow=off  InputSameDT=off
  Manual Switch3_EnableFlag : Constant  Value=FAULT_13_FGSupplyPressOscillation_enable
  Manual Switch3_Switch : Switch  Threshold=0.5  SaturateOnIntegerOverflow=off  InputSameDT=off
  Manual Switch4_EnableFlag : Constant  Value=FAULT_12_FuelSupplyPressDrop_enable
  Manual Switch4_Switch : Switch  Threshold=0.5  SaturateOnIntegerOverflow=off  InputSameDT=off
  Manual Switch5_EnableFlag : Constant  Value=FAULT_11_FuelPumpDegradation_enable
  Manual Switch5_Switch : Switch  Threshold=0.5  SaturateOnIntegerOverflow=off  InputSameDT=off
  Manual Switch6_EnableFlag : Constant  Value=FAULT_07_FuelPrssRegulatorStuck_enable
  Manual Switch6_Switch : Switch  Threshold=0.5  SaturateOnIntegerOverflow=off  InputSameDT=off
  Manual Switch7_EnableFlag : Constant  Value=FAULT_16_FuelValveLeak_enable
  Manual Switch7_Switch : Switch  Threshold=0.5  SaturateOnIntegerOverflow=off  InputSameDT=off
  Manual Switch8_EnableFlag : Constant  Value=FAULT_08_FuelValveLeakage_enable
  Manual Switch8_Switch : Switch  Threshold=0.5  SaturateOnIntegerOverflow=off  InputSameDT=off
  Prss_FG_Aftr_MCV_PT204_kPa : ToWorkspace  VariableName=Prss_FG_Aftr_MCV_PT204_kPa  SampleTime=0.2
  Subsystem1 : Subsystem
  FG Temp (oC) : Outport
  FG Flow @bur (kg/s) : Outport  Port=2
  FG pr @bur (kPa) : Outport  Port=3
  FG skid inlet prss (kPa) : Outport  Port=4
  tag scope: FG_flow=global
  wires:
  Subsystem1/2(skid temp) -> CV model chamber 2/3(FG temp.)
  " Memory "/1 -> Subsystem1/3(FG flow)
  Subsystem1/1(" FG skid inlet prss") -> CV model chamber 2/2(Skid inlet prss), Prss_FG_Aftr_MCV_PT204_kPa/1, FG skid inlet prss (kPa)/1
  FG temp./1 -> Subsystem1/2(FG temp.), FG Temp (oC)/1
  CV model chamber 2/1(FG pr @bur) -> FG pr @bur (kPa)/1
  FG CV pos (%) chmb1/1 -> CV model chamber 2/1(FG valve pos.)
  CV model chamber 2/2(FG flow) -> FAULT_16_FuelValveLeak/1(FG flow), Manual Switch7_Switch/3
  main FG line prss/1 -> FAULT_07_FuelPrssRegulatorStuck/1(main FG line prss), Manual Switch6_Switch/3
  FAULT_09_FuelContamination/1(Out1) -> Manual Switch1_Switch/1
  Manual Switch1_EnableFlag/1 -> Manual Switch1_Switch/2
  Manual Switch1_Switch/1 -> FAULT_08_FuelValveLeakage/1(In1), Manual Switch8_Switch/3
  FAULT_10_FuelLineBlockage/1(Out1) -> Manual Switch2_Switch/1
  Manual Switch2_EnableFlag/1 -> Manual Switch2_Switch/2
  Manual Switch2_Switch/1 -> [FG_flow], " Memory "/1, FG Flow @bur (kg/s)/1
  FAULT_13_FGSupplyPressOscillation/1(Out1) -> Manual Switch3_Switch/1
  Manual Switch3_EnableFlag/1 -> Manual Switch3_Switch/2
  Manual Switch3_Switch/1 -> Subsystem1/1(gas prss)
  FAULT_12_FuelSupplyPressDrop/1(Out1) -> Manual Switch4_Switch/1
  Manual Switch4_EnableFlag/1 -> Manual Switch4_Switch/2
  Manual Switch4_Switch/1 -> Manual Switch3_Switch/3, FAULT_13_FGSupplyPressOscillation/1(In1)
  FAULT_11_FuelPumpDegradation/1(Out1) -> Manual Switch5_Switch/1
  Manual Switch5_EnableFlag/1 -> Manual Switch5_Switch/2
  Manual Switch5_Switch/1 -> Manual Switch4_Switch/3, FAULT_12_FuelSupplyPressDrop/1(In1)
  FAULT_07_FuelPrssRegulatorStuck/1(Out1) -> Manual Switch6_Switch/1
  Manual Switch6_EnableFlag/1 -> Manual Switch6_Switch/2
  Manual Switch6_Switch/1 -> Manual Switch5_Switch/3, FAULT_11_FuelPumpDegradation/1(In1)
  FAULT_16_FuelValveLeak/1(Out1) -> Manual Switch7_Switch/1
  Manual Switch7_EnableFlag/1 -> Manual Switch7_Switch/2
  Manual Switch7_Switch/1 -> Manual Switch1_Switch/3, FAULT_09_FuelContamination/1(In1)
  FAULT_08_FuelValveLeakage/1(Out1) -> Manual Switch8_Switch/1
  Manual Switch8_EnableFlag/1 -> Manual Switch8_Switch/2
  Manual Switch8_Switch/1 -> Manual Switch2_Switch/3, FAULT_10_FuelLineBlockage/1(In1)

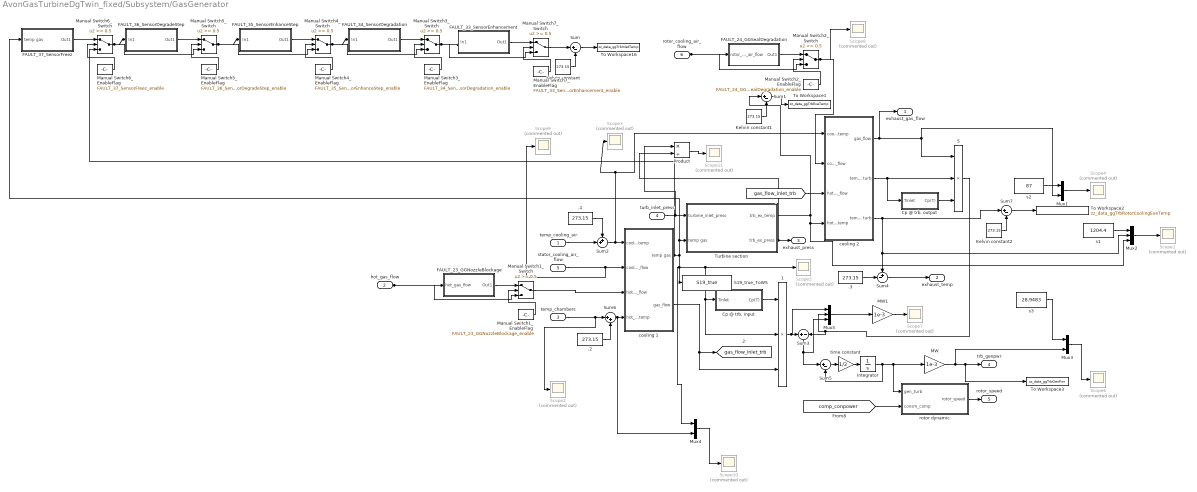
== system AvonGasTurbineDgTwin_fixed/Subsystem/GasGenerator ==
  temp_cooling_air : Inport
  hot_gas_flow : Inport  Port=2
  temp_chambers : Inport  Port=3
  turb_inlet_press : Inport  Port=4
  stator_cooling_air_flow : Inport  Port=5
  rotor_cooling_air_flow : Inport  Port=6
  "    .1" : Constant  Value=273.15
  "    .2" : Constant  Value=273.15
  "    .3" : Constant  Value=273.15
  " 1" : Product  Inputs=3  RndMeth=Zero
  " 5" : Product  Inputs=3  RndMeth=Zero
  Cp @ trb. input : Subsystem
  Cp @ trb. output : Subsystem
  FAULT_23_GGNozzleBlockage : Subsystem
  FAULT_24_GGSealDegradation : Subsystem
  FAULT_33_SensorEnhancement : Subsystem
  FAULT_34_SensorDegradation : Subsystem
  FAULT_35_SensorEnhanceStep : Subsystem
  FAULT_36_SensorDegradeStep : Subsystem
  FAULT_37_SensorFreez : Subsystem
  Integrator : Integrator  InitialCondition=13500  LimitOutput=on  UpperSaturationLimit=34000  LowerSaturationLimit=10
  Kelvin constant : Constant  Value=273.15
  Kelvin constant1 : Constant  Value=273.15
  Kelvin constant2 : Constant  Value=273.15
  MW : Gain  Gain=1e-3
  MW1 : Gain  Gain=1e-3
  Manual Switch1_EnableFlag : Constant  Value=FAULT_23_GGNozzleBlockage_enable
  Manual Switch1_Switch : Switch  Threshold=0.5  SaturateOnIntegerOverflow=off  InputSameDT=off
  Manual Switch2_EnableFlag : Constant  Value=FAULT_24_GGSealDegradation_enable
  Manual Switch2_Switch : Switch  Threshold=0.5  SaturateOnIntegerOverflow=off  InputSameDT=off
  Manual Switch3_EnableFlag : Constant  Value=FAULT_34_SensorDegradation_enable
  Manual Switch3_Switch : Switch  Threshold=0.5  SaturateOnIntegerOverflow=off  InputSameDT=off
  Manual Switch4_EnableFlag : Constant  Value=FAULT_35_SensorEnhanceStep_enable
  Manual Switch4_Switch : Switch  Threshold=0.5  SaturateOnIntegerOverflow=off  InputSameDT=off
  Manual Switch5_EnableFlag : Constant  Value=FAULT_36_SensorDegradeStep_enable
  Manual Switch5_Switch : Switch  Threshold=0.5  SaturateOnIntegerOverflow=off  InputSameDT=off
  Manual Switch6_EnableFlag : Constant  Value=FAULT_37_SensorFreez_enable
  Manual Switch6_Switch : Switch  Threshold=0.5  SaturateOnIntegerOverflow=off  InputSameDT=off
  Manual Switch7_EnableFlag : Constant  Value=FAULT_33_SensorEnhancement_enable
  Manual Switch7_Switch : Switch  Threshold=0.5  SaturateOnIntegerOverflow=off  InputSameDT=off
  Mux1 : Mux  Inputs=2
  Mux2 : Mux  Inputs=3
  Mux3 : Mux  Inputs=2
  Mux4 : Mux  Inputs=2
  Mux5 : Mux  Inputs=3
  Product : Product  Inputs=*/
  S19_true_ToWS : ToWorkspace  VariableName=S19_true  SampleTime=-1
  Scope{1..11} (11 alike) : Scope  Commented=on
  Sum{,1,5,7} (4 alike) : Sum  Inputs=|+-
  Sum2 : Sum  Inputs=++|
  Sum3 : Sum  Inputs=+-
  Sum4 : Sum  Inputs=+-|
  Sum6 : Sum  Inputs=|++
  To Workspace1 : ToWorkspace  VariableName=zz_data_ggTrbExeTemp  SampleTime=0.2
  To Workspace16 : ToWorkspace  VariableName=zz_data_ggTrbInletTemp  SampleTime=0.2
  To Workspace2 : ToWorkspace  VariableName=zz_data_ggTrbRotorCoolingExeTemp  SampleTime=0.2
  To Workspace3 : ToWorkspace  VariableName=zz_data_ggTrbGenPwr  SampleTime=0.2
  Turbine section : Subsystem
  cooling 1 : Subsystem
  cooling 2 : Subsystem
  "rotor dynamic " : Subsystem
  s1 : Constant  Value=1204.4
  s2 : Constant  Value=87
  s3 : Constant  Value=28.9483
  time constant : Gain  Gain=1/2
  exhaust_gas_flow : Outport
  exhaust_temp : Outport  Port=2
  exhaust_press : Outport  Port=3
  trb_genpwr : Outport  Port=4
  rotor_speed : Outport  Port=5
  tag scope: gas_flow_inlet_trb=global
  wires:
  Sum2/1 -> cooling 1/1(cooling_air_temp), cooling 2/1(cooling_air_temp), Scope3/1
  " 1"/1 -> Mux5/1, Sum3/1
  Sum5/1 -> time constant/1
  time constant/1 -> Integrator/1
  [gas_flow_inlet_trb] -> cooling 2/3(hot_gas_flow)
  Cp @ trb. input/1(Cp(T)) -> " 1"/1
  Turbine section/1(trb_ex_temp) -> Sum1/1, Mux2/3, cooling 2/4(hot_gas_temp)
  cooling 2/3(temp exh turb) -> Sum7/1, Mux2/2, Sum4/1
  Cp @ trb. output/1(Cp(T)) -> " 5"/3
  " 5"/1 -> Sum3/2, Mux5/2
  cooling 1/2(gas_flow) -> " 1"/3, [gas_flow_inlet_trb]
  Sum3/1 -> Mux5/3, Sum5/1
  Mux1/1 -> Scope4/1
  s2/1 -> Mux1/1
  cooling 2/1(gas_flow) -> " 5"/1, Mux1/2, exhaust_gas_flow/1
  Mux2/1 -> Scope1/1
  s1/1 -> Mux2/1
  "    .1"/1 -> Sum2/1
  temp_cooling_air/1 -> Sum2/2
  "    .2"/1 -> Sum6/2
  temp_chambers/1 -> Scope2/1, Sum6/1
  Sum4/1 -> exhaust_temp/1
  "    .3"/1 -> Sum4/2
  turb_inlet_press/1 -> Product/1, Turbine section/1(turbine_inlet_press)
  Mux3/1 -> Scope6/1
  s3/1 -> Mux3/1
  Integrator/1 -> "rotor dynamic "/1(gen_turb), MW/1, Sum5/2
  cooling 2/2(temp turb) -> Cp @ trb. output/1(Tinlet), " 5"/2
  Turbine section/2(trb_ex_press) -> exhaust_press/1, Product/2
  MW/1 -> Mux3/2, To Workspace3/1, trb_genpwr/1
  [comp_conpower] -> "rotor dynamic "/2(consm_comp)
  "rotor dynamic "/1(rotor_speed) -> rotor_speed/1
  stator_cooling_air_flow/1 -> cooling 1/2(cooling_air_flow), Scope9/1
  Mux4/1 -> Scope10/1
  cooling 1/1(temp gas) -> Turbine section/2(temp gas), FAULT_37_SensorFreez/1(temp gas), Cp @ trb. input/1(Tinlet), " 1"/2, Scope5/1, Mux4/1, Manual Switch6_Switch/3, S19_true_ToWS/1
  Sum6/1 -> Mux4/2, cooling 1/4(hot_gas_temp)
  Mux5/1 -> MW1/1
  MW1/1 -> Scope7/1
  Product/1 -> Scope11/1
  hot_gas_flow/1 -> FAULT_23_GGNozzleBlockage/1(hot_gas_flow), Manual Switch1_Switch/3
  rotor_cooling_air_flow/1 -> FAULT_24_GGSealDegradation/1(rotor_cooling_air_flow), Manual Switch2_Switch/3
  Kelvin constant/1 -> Sum/2
  Sum/1 -> To Workspace16/1
  Kelvin constant1/1 -> Sum1/2
  Sum1/1 -> To Workspace1/1
  Kelvin constant2/1 -> Sum7/2
  Sum7/1 -> To Workspace2/1
  FAULT_23_GGNozzleBlockage/1(Out1) -> Manual Switch1_Switch/1
  Manual Switch1_EnableFlag/1 -> Manual Switch1_Switch/2
  Manual Switch1_Switch/1 -> cooling 1/3(hot_gas_flow)
  FAULT_24_GGSealDegradation/1(Out1) -> Manual Switch2_Switch/1
  Manual Switch2_EnableFlag/1 -> Manual Switch2_Switch/2
  Manual Switch2_Switch/1 -> Scope8/1, cooling 2/2(cooling_air_flow)
  FAULT_34_SensorDegradation/1(Out1) -> Manual Switch3_Switch/1
  Manual Switch3_EnableFlag/1 -> Manual Switch3_Switch/2
  Manual Switch3_Switch/1 -> FAULT_33_SensorEnhancement/1(In1), Manual Switch7_Switch/3
  FAULT_35_SensorEnhanceStep/1(Out1) -> Manual Switch4_Switch/1
  Manual Switch4_EnableFlag/1 -> Manual Switch4_Switch/2
  Manual Switch4_Switch/1 -> Manual Switch3_Switch/3, FAULT_34_SensorDegradation/1(In1)
  FAULT_36_SensorDegradeStep/1(Out1) -> Manual Switch5_Switch/1
  Manual Switch5_EnableFlag/1 -> Manual Switch5_Switch/2
  Manual Switch5_Switch/1 -> Manual Switch4_Switch/3, FAULT_35_SensorEnhanceStep/1(In1)
  FAULT_37_SensorFreez/1(Out1) -> Manual Switch6_Switch/1
  Manual Switch6_EnableFlag/1 -> Manual Switch6_Switch/2
  Manual Switch6_Switch/1 -> Manual Switch5_Switch/3, FAULT_36_SensorDegradeStep/1(In1)
  FAULT_33_SensorEnhancement/1(Out1) -> Manual Switch7_Switch/1
  Manual Switch7_EnableFlag/1 -> Manual Switch7_Switch/2
  Manual Switch7_Switch/1 -> Sum/1

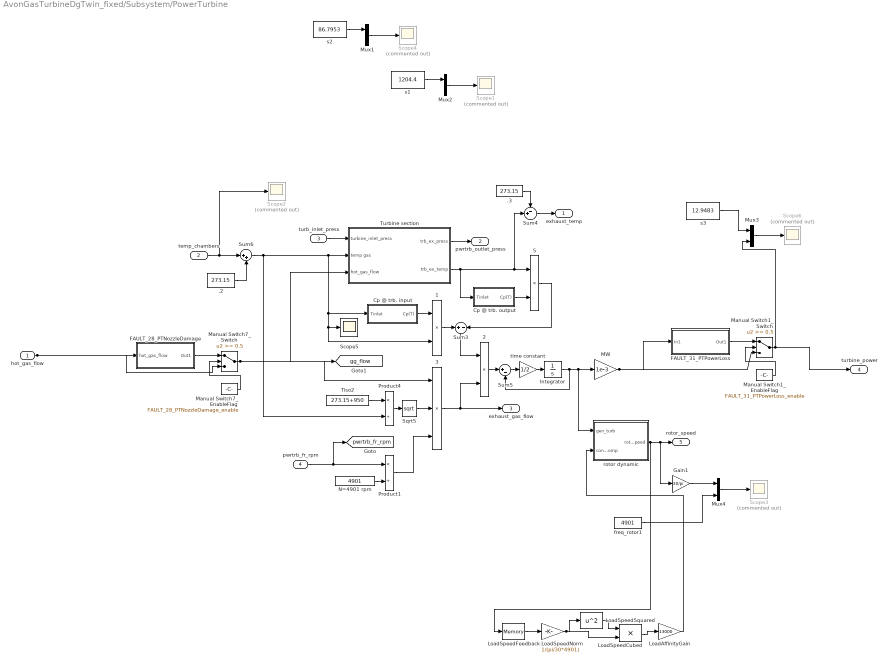
== system AvonGasTurbineDgTwin_fixed/Subsystem/PowerTurbine ==
  hot_gas_flow : Inport
  temp_chambers : Inport  Port=2
  turb_inlet_press : Inport  Port=3
  pwrtrb_fr_rpm : Inport  Port=4
  "    .2" : Constant  Value=273.15
  "    .3" : Constant  Value=273.15
  " 1" : Product  RndMeth=Zero
  " 2" : Product  RndMeth=Zero
  " 3" : Product  Inputs=3  RndMeth=Zero
  " 5" : Product  RndMeth=Zero
  Cp @ trb. input : Subsystem
  Cp @ trb. output : Subsystem
  FAULT_28_PTNozzleDamage : Subsystem
  FAULT_31_PTPowerLoss : Subsystem
  Gain1 : Gain  Gain=30/pi
  Integrator : Integrator  InitialCondition=13000  LimitOutput=on  UpperSaturationLimit=20000  LowerSaturationLimit=1
  LoadAffinityGain : Gain  Gain=13000
  LoadSpeedCubed : Product  Inputs=**
  LoadSpeedFeedback : Memory  InitialCondition=pi/30*4901
  LoadSpeedNorm : Gain  Gain=1/(pi/30*4901)
  LoadSpeedSquared : Math  Operator=square
  MW : Gain  Gain=1e-3
  Manual Switch1_EnableFlag : Constant  Value=FAULT_31_PTPowerLoss_enable
  Manual Switch1_Switch : Switch  Threshold=0.5  SaturateOnIntegerOverflow=off  InputSameDT=off
  Manual Switch7_EnableFlag : Constant  Value=FAULT_28_PTNozzleDamage_enable
  Manual Switch7_Switch : Switch  Threshold=0.5  SaturateOnIntegerOverflow=off  InputSameDT=off
  Mux1 : Mux  Inputs=2
  Mux2 : Mux  Inputs=3
  Mux3 : Mux  Inputs=2
  Mux4 : Mux  Inputs=2
  N=4901 rpm : Constant  Value=4901
  Product1 : Product  Inputs=*/  RndMeth=Zero
  Product4 : Product  Inputs=*/  RndMeth=Zero
  Scope{1..4,6} (5 alike) : Scope  Commented=on
  Scope5 : Scope
  Sqrt5 : Sqrt
  Sum3 : Sum  Inputs=+-
  Sum4 : Sum  Inputs=-+|
  Sum5 : Sum  Inputs=|+-
  Sum6 : Sum  Inputs=|++
  Tiso2 : Constant  Value=273.15+950
  Turbine section : Subsystem
  freq_rotor1 : Constant  Value=4901
  rotor dynamic : Subsystem
  s1 : Constant  Value=1204.4
  s2 : Constant  Value=86.7953
  s3 : Constant  Value=12.9483
  time constant : Gain  Gain=1/2
  exhaust_temp : Outport
  pwrtrb_outlet_press : Outport  Port=2
  exhaust_gas_flow : Outport  Port=3
  turbine_power : Outport  Port=4
  rotor_speed : Outport  Port=5
  tag scope: gg_flow=global, pwrtrb_fr_rpm=global
  wires:
  Turbine section/2(trb_ex_temp) -> " 5"/1, Sum4/2, Cp @ trb. output/1(Tinlet)
  s3/1 -> Mux3/1
  Mux3/1 -> Scope6/1
  turb_inlet_press/1 -> Turbine section/1(turbine_inlet_press)
  "    .3"/1 -> Sum4/1
  Sum4/1 -> exhaust_temp/1
  temp_chambers/1 -> Scope2/1, Sum6/1
  "    .2"/1 -> Sum6/2
  s1/1 -> Mux2/1
  Mux2/1 -> Scope1/1
  s2/1 -> Mux1/1
  Mux1/1 -> Scope4/1
  " 2"/1 -> Sum5/1
  " 5"/1 -> Sum3/2
  Cp @ trb. output/1(Cp(T)) -> " 5"/2
  Cp @ trb. input/1(Cp(T)) -> " 1"/1
  time constant/1 -> Integrator/1
  Sum5/1 -> time constant/1
  " 1"/1 -> Sum3/1
  Sum3/1 -> " 2"/1
  Tiso2/1 -> Product4/1
  Sum6/1 -> Product4/2, Cp @ trb. input/1(Tinlet), " 1"/2, Scope5/1, Turbine section/2(temp gas)
  Product4/1 -> Sqrt5/1
  N=4901 rpm/1 -> Product1/2
  pwrtrb_fr_rpm/1 -> [pwrtrb_fr_rpm], Product1/1
  Product1/1 -> " 3"/3
  Sqrt5/1 -> " 3"/2
  " 3"/1 -> exhaust_gas_flow/1, " 2"/2
  Turbine section/1(trb_ex_press) -> pwrtrb_outlet_press/1
  rotor dynamic/1(rotor_speed) -> Gain1/1, rotor_speed/1, LoadSpeedFeedback/1
  Integrator/1 -> Sum5/2, MW/1, rotor dynamic/1(gen_turb)
  Mux4/1 -> Scope3/1
  freq_rotor1/1 -> Mux4/2
  Gain1/1 -> Mux4/1
  hot_gas_flow/1 -> FAULT_28_PTNozzleDamage/1(hot_gas_flow), Manual Switch7_Switch/3
  MW/1 -> FAULT_31_PTPowerLoss/1(In1), Manual Switch1_Switch/3
  LoadSpeedFeedback/1 -> LoadSpeedNorm/1
  LoadSpeedNorm/1 -> LoadSpeedSquared/1, LoadSpeedCubed/2
  LoadSpeedSquared/1 -> LoadSpeedCubed/1
  LoadSpeedCubed/1 -> LoadAffinityGain/1
  LoadAffinityGain/1 -> rotor dynamic/2(consm_comp)
  FAULT_31_PTPowerLoss/1(Out1) -> Manual Switch1_Switch/1
  Manual Switch1_EnableFlag/1 -> Manual Switch1_Switch/2
  Manual Switch1_Switch/1 -> turbine_power/1, Mux3/2
  FAULT_28_PTNozzleDamage/1(Out1) -> Manual Switch7_Switch/1
  Manual Switch7_EnableFlag/1 -> Manual Switch7_Switch/2
  Manual Switch7_Switch/1 -> [gg_flow], Turbine section/3(hot_gas_flow), " 3"/1
